simulink library "Main_Controller_Lib"  (R2025a)
settings: Solver=ode45  StartTime=0.0  StopTime=10.0  RelTol=1e-3  EnableMultiTasking=on
undefined symbols (not defined in the file): Actuator_Lookup, radps2rpm
libraries: Turbine_State_Machine_Lib x1
Description:
  | Copyright 2009-2025 The MathWorks, Inc. MathWorks, Inc.
settings Model: Creator=smiller  LastModifiedBy=smiller
settings SolverCC: AlgebraicLoopSolver=TrustRegion
settings DataIOCC: LimitDataPoints=on  SaveFormat=Array  SignalLoggingSaveFormat=ModelDataLogs  ReturnWorkspaceOutputs=off
settings OptimizationCC: ReuseModelBlockBuffer=off  ExpressionDepthLimit=2147483647.0  LifeSpan=inf
settings DebuggingCC: UnderspecifiedInitializationDetection=Classic  MergeDetectMultiDrivingBlocksExec=none  SolverPrmCheckMsg=warning  FcnCallInpInsideContextMsg=warning  UnconnectedInputMsg=warning  UnconnectedOutputMsg=warning  UnconnectedLineMsg=warning  AllowSymbolicDim=off  StateNameClashWarn=warning  PregeneratedLibrarySubsystemCodeDiagnostic=none  SFUnexpectedBacktrackingDiag=warning  SFNoUnconditionalDefaultTransitionDiag=warning  SFExecutionAtInitializationDiag=none  ArithmeticOperatorsInVariantConditions=warning
settings HardwareCC: ProdBitPerPointer=32.0  ProdBitPerSizeT=32.0  ProdBitPerPtrDiffT=32.0  ProdLargestAtomicFloat=None  ProdIntDivRoundTo=Undefined  ProdEndianess=Unspecified  ProdWordSize=32.0  ProdHWDeviceType=32-bit Generic
settings ModelReferenceCC: EnableRefExpFcnMdlSchedulingChecks=on  PropagateSignalLabelsOutOfModel=off
settings SFSimCC: SimUseLocalCustomCode=off  CustomCodeUndefinedFunction=UseInterfaceOnly
settings RTWCC: RTWUseLocalCustomCode=off  GPUComputeCapability=3.5  DLArmComputeVersion=19.05
settings CodeAppCC: StateflowObjectComments=on
settings GRTTargetCC: TargetLangStandard=C89/C90 (ANSI)  CombineOutputUpdateFcns=off  GRTInterface=on
settings ConfigComp: CovMetricSettings=dw  CovSaveCumulativeToWorkspaceVar=on  CovSaveSingleToWorkspaceVar=on  CovExternalEMLEnable=off  CovSFcnEnable=off

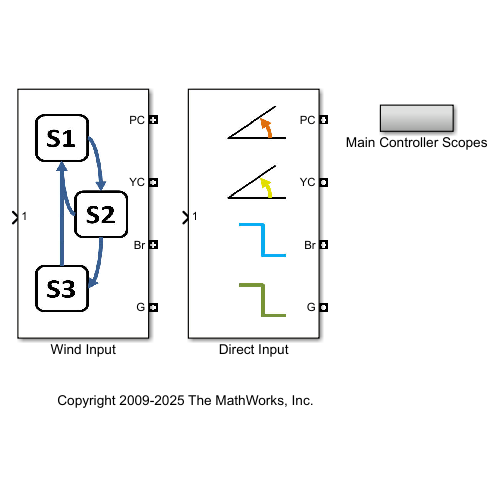
[thumbnail: Simulink's stored preview of the top-level diagram]
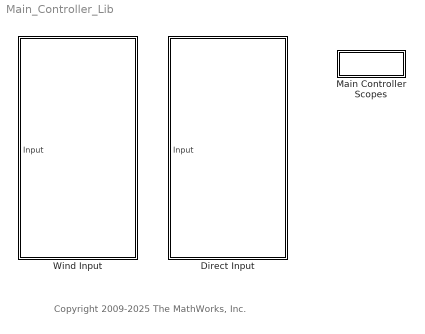
== system Main_Controller_Lib ==
  note: Copyright 2009-2025 The MathWorks, Inc.
  Direct Input : Subsystem
      mask Display: image('Main_Controller_Direct_Input_IMAGE.jpg');
  Main Controller Scopes : Subsystem
  Wind Input : Subsystem
      mask Display: image('Main_Controller_Wind_Input_IMAGE.jpg');

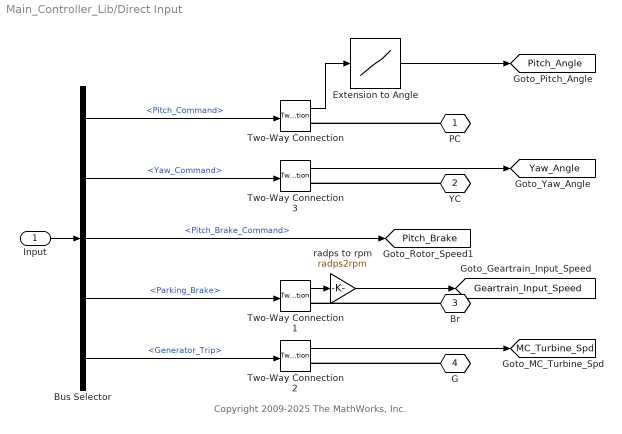
== system Main_Controller_Lib/Direct Input ==
  note: Copyright 2009-2025 The MathWorks, Inc.
  Input : Inport
  Bus Selector : BusSelector  OutputSignals=Pitch_Command,Yaw_Command,Pitch_Brake_Command,Parking_Brake,Generator_Trip
  Extension to Angle : Lookup  InputValues=Actuator_Lookup.extension  Table=Actuator_Lookup.angle  SaturateOnIntegerOverflow=off
  Two-Way Connection{,1..3} (4 alike) : TwoWayConnection
  radps to rpm : Gain  Gain=radps2rpm
  PC : PMIOPort  Tag=PMCPort  Side=Right
  YC : PMIOPort  Tag=PMCPort  Port=2  Side=Right
  Br : PMIOPort  Tag=PMCPort  Port=3  Side=Right
  G : PMIOPort  Tag=PMCPort  Port=4  Side=Right
  tag scope: Geartrain_Input_Speed=global, MC_Turbine_Spd=global, Pitch_Angle=global, Pitch_Brake=global, Yaw_Angle=global
  wires:
  Bus Selector/5 -> Two-Way Connection2/1  "<Generator_Trip>"
  Bus Selector/4 -> Two-Way Connection1/1  "<Parking_Brake>"
  Bus Selector/3 -> [Pitch_Brake]  "<Pitch_Brake_Command>"
  radps to rpm/1 -> [Geartrain_Input_Speed]
  Bus Selector/2 -> Two-Way Connection3/1  "<Yaw_Command>"
  Two-Way Connection3/1 -> [Yaw_Angle]
  Two-Way Connection1/1 -> radps to rpm/1
  Bus Selector/1 -> Two-Way Connection/1  "<Pitch_Command>"
  Two-Way Connection/1 -> Extension to Angle/1
  Extension to Angle/1 -> [Pitch_Angle]
  Two-Way Connection2/1 -> [MC_Turbine_Spd]
  Input/1 -> Bus Selector/1
  connections:
  PC/RConn1 -- Two-Way Connection/RConn1
  Br/RConn1 -- Two-Way Connection1/RConn1
  G/RConn1 -- Two-Way Connection2/RConn1
  YC/RConn1 -- Two-Way Connection3/RConn1

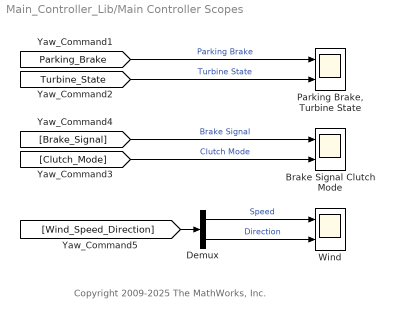
== system Main_Controller_Lib/Main Controller Scopes ==
  note: Copyright 2009-2025 The MathWorks, Inc.
  Brake Signal Clutch Mode : Scope  NumInputPorts=2
      settings: TimeSpan=80  ActiveDisplayYMinimum=-1  ActiveDisplayYMaximum=1  DataLoggingVariableName=ScopeData9
  Demux : Demux  Outputs=2
  "Parking Brake, Turbine State" : Scope  NumInputPorts=2
      settings: TimeSpan=80  ActiveDisplayYMinimum=0  ActiveDisplayYMaximum=1  DataLoggingVariableName=ScopeData7
  Wind : Scope  NumInputPorts=2
      settings: TimeSpan=80  ActiveDisplayYMinimum=0  ActiveDisplayYMaximum=20  DataLoggingVariableName=Wind_Turbine_Wind_DATA
  wires:
  Demux/2 -> Wind/2  "Direction"
  Demux/1 -> Wind/1  "Speed"
  [Wind_Speed_Direction] -> Demux/1
  [Clutch_Mode] -> Brake Signal Clutch Mode/2  "Clutch Mode"
  [Brake_Signal] -> Brake Signal Clutch Mode/1  "Brake Signal"
  [Turbine_State] -> "Parking Brake, Turbine State"/2  "Turbine State"
  [Parking_Brake] -> "Parking Brake, Turbine State"/1  "Parking Brake"

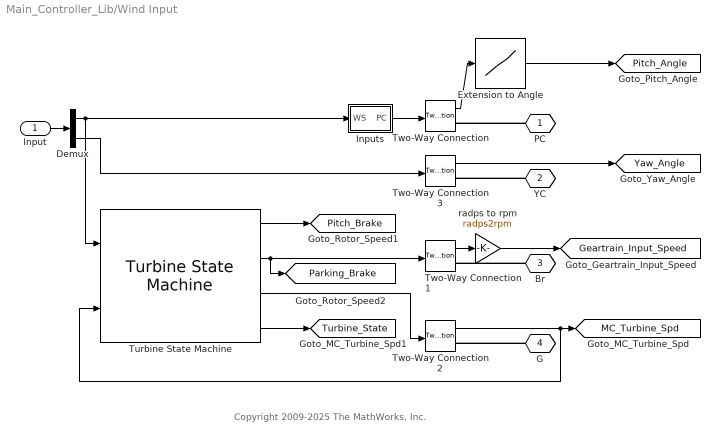
== system Main_Controller_Lib/Wind Input ==
  note: Copyright 2009-2025 The MathWorks, Inc.
  Input : Inport
  Demux : Demux  Outputs=2
  Extension to Angle : Lookup  InputValues=Actuator_Lookup.extension  Table=Actuator_Lookup.angle  SaturateOnIntegerOverflow=off
  Inputs : Subsystem
  Turbine State Machine : Turbine_State_Machine_Lib/Turbine State Machine  SystemSampleTime=-1  VariantActivationTime=update diagram  EmptyChoice=off  PassThrough=off  PassThroughVariantControl=(default)  EmptyChoiceVariantControl=(default)  AllowFlexibleInterface=on  Latency=0  AutoFrameSizeCalculation=off
  Two-Way Connection{,1..3} (4 alike) : TwoWayConnection
  radps to rpm : Gain  Gain=radps2rpm
  PC : PMIOPort  Tag=PMCPort  Side=Right
  YC : PMIOPort  Tag=PMCPort  Port=2  Side=Right
  Br : PMIOPort  Tag=PMCPort  Port=3  Side=Right
  G : PMIOPort  Tag=PMCPort  Port=4  Side=Right
  tag scope: Geartrain_Input_Speed=global, MC_Turbine_Spd=global, Parking_Brake=global, Pitch_Angle=global, Pitch_Brake=global, Turbine_State=global, Yaw_Angle=global
  wires:
  Inputs/1(PC) -> Two-Way Connection/1
  radps to rpm/1 -> [Geartrain_Input_Speed]
  Demux/2 -> Two-Way Connection3/1
  Two-Way Connection3/1 -> [Yaw_Angle]
  Two-Way Connection1/1 -> radps to rpm/1
  Demux/1 -> Inputs/1(WS), Turbine State Machine/1
  Two-Way Connection/1 -> Extension to Angle/1
  Extension to Angle/1 -> [Pitch_Angle]
  Two-Way Connection2/1 -> [MC_Turbine_Spd], Turbine State Machine/2
  Input/1 -> Demux/1
  Turbine State Machine/3 -> Two-Way Connection2/1
  Turbine State Machine/1 -> [Pitch_Brake]
  Turbine State Machine/2 -> Two-Way Connection1/1, [Parking_Brake]
  Turbine State Machine/4 -> [Turbine_State]
  connections:
  PC/RConn1 -- Two-Way Connection/RConn1
  Br/RConn1 -- Two-Way Connection1/RConn1
  G/RConn1 -- Two-Way Connection2/RConn1
  YC/RConn1 -- Two-Way Connection3/RConn1

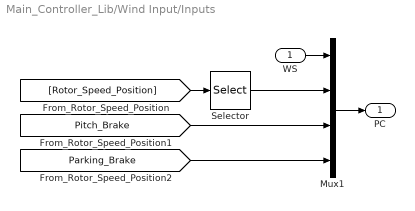
== system Main_Controller_Lib/Wind Input/Inputs ==
  WS : Inport
  Mux1 : Mux
  Selector : Selector  InputPortWidth=2  IndexOptions=Index vector (dialog)  Indices=[2]  OutputSizes=1
  PC : Outport  VectorParamsAs1DForOutWhenUnconnected=off
  wires:
  [Rotor_Speed_Position] -> Selector/1
  Selector/1 -> Mux1/2
  WS/1 -> Mux1/1
  Mux1/1 -> PC/1
  [Pitch_Brake] -> Mux1/3
  [Parking_Brake] -> Mux1/4
